simulink model "Simulink_Simulation"  (R2025a)
settings: Solver=VariableStepAuto  StartTime=0.0  StopTime=10.0  RelTol=1e-3
settings Model: Creator=Pioneer  LastModifiedBy=Pioneer

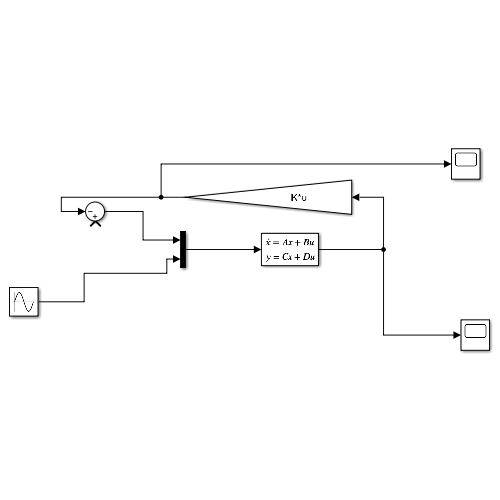
[thumbnail: Simulink's stored preview of the top-level diagram]
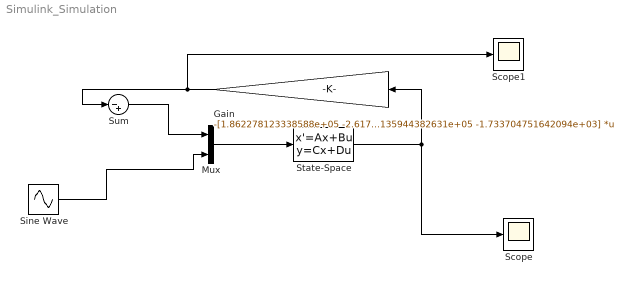
== system Simulink_Simulation ==
  Gain : Gain  Gain="-[1.862278123338588e+05\t-2.617409040772817e+02\t-1.201135944382631e+05\t-1.733704751642094e+03]"  Multiplication=Matrix(K*u)
  Mux : Mux  Inputs=2
  Scope : Scope
      settings: ActiveDisplayYMinimum=-267.80393302674116  ActiveDisplayYMaximum=267.84148545676885
  Scope1 : Scope
      settings: ActiveDisplayYMinimum=-1.4145659019136902  ActiveDisplayYMaximum=1.6690438045484528
  Sine Wave : Sin  SampleTime=0
  State-Space : StateSpace  A=|  B=|  C=eye(4)  D=zeros(4,2)  InitialCondition=0
      A=|
      | [0  1   0   0;
      |      -(2000*300)/(300*45)  0  ((2000/300)*((2000/300)+(2000/45)+(300/45)))-(22500/300)   -2000/300;
      |       300/45  0   -((2000/300)+(2000/45)+(300/45))   1;
      |       200000/45  0  -((22500/300)+(22500/45)+(200000/45))   0]
      B=|
      | [ 0     0;
      |       (1/300)     (2000*300)/(300*45);
      |       0    -300/45;
      |      ((1/300)+(1/45))    -200000/45]
  Sum : Sum  Inputs=|-+
  wires:
  Mux/1 -> State-Space/1
  State-Space/1 -> Gain/1, Scope/1
  Sine Wave/1 -> Mux/2
  Gain/1 -> Scope1/1, Sum/1
  Sum/1 -> Mux/1
